simulink model "FSI02"  (R2024b)
settings: Solver=ode4  StartTime=0.0  StopTime=4  FixedStep=0.5  RelTol=1e-3
values from neighbouring files (symbols this model uses):
  x1 = 1    [FSI02WS.m]
settings Model: Creator=fmiro  LastModifiedBy=fmiro

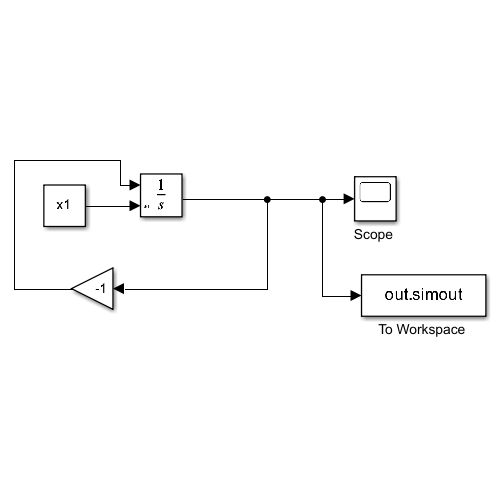
[thumbnail: Simulink's stored preview of the top-level diagram]
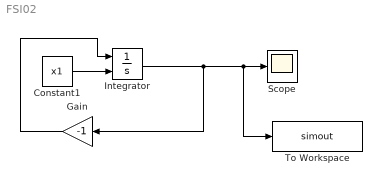
== system FSI02 ==
  Constant1 : Constant  Value=x1
  Gain : Gain  Gain=-1
  Integrator : Integrator  InitialConditionSource=external
  "Scope " : Scope
  "To Workspace " : ToWorkspace  VariableName=simout  SaveFormat=Structure  SampleTime=-1
      settings: Save2DSignal=2-D array (concatenate along first dimension)
  wires:
  Integrator/1 -> "To Workspace "/1, "Scope "/1, Gain/1
  Constant1/1 -> Integrator/2
  Gain/1 -> Integrator/1
